simulink model "tp_thyr_rect_sm"  (R2026a)
settings: Solver=daessc  StopTime=simlength  FixedStep=Ts  MaxStep=Ts  RelTol=Ts  AbsTol=Ts  EnableMultiTasking=on
values from neighbouring files (symbols this model uses):
  I_FS = Iout_dc_nom * margin_factor    (= 103.5)    [init_model.m]
  kgrid = 1    [init_model.m]
  LFu_dc = 1.2e-3    (= 0.0012)    [init_model.m]
  pll_i1 = 80    [init_model.m]
  pll_p = 1    [init_model.m]
  RLFu_dc = 2e-4    (= 0.0002)    [init_model.m]
  Rload = 1.2/4    (= 0.3)    [init_model.m]
  Tc = 1e-5    (= 1e-05)    [init_model.m]
  Tcontrol_rect = tPWM_RECT    (= 0.0002)    [init_model.m]
  Ts = Tc/1    (= 1e-05)    [init_model.m]
  V_FS = Vout_dc_nom * margin_factor    (= 391)    [init_model.m]
  Vnom_ac_adc = 400/sqrt(3)*sqrt(2)    [init_model.m]
  Vphase1 = Vline1/sqrt(3)    [init_model.m]
  w_grid = f_grid*2*pi    (= 314.159265359)    [init_model.m]
undefined symbols (not defined in the file or in its folder): magnitude
libraries: fl_lib x248, nesl_utility x39, ee_lib x28
(part 1 of 5)
settings Model: Creator=LTNBDA  LastModifiedBy=dbagn
settings SolverCC: ZeroCrossControl=EnableAll  ZeroCrossAlgorithm=Adaptive  SolverResetMethod=Robust
settings DataIOCC: MaxDataPoints=1  SignalLoggingSaveFormat=ModelDataLogs
settings OptimizationCC: InitFltsAndDblsToZero=on  EfficientMapNaN2IntZero=off
settings DebuggingCC: SaveWithParameterizedLinksMsg=none  UnderspecifiedInitializationDetection=Classic  SignalResolutionControl=TryResolveAllWithWarning  MultiTaskDSMMsg=warning  MultiTaskCondExecSysMsg=none
settings HardwareCC: ProdBitPerLong=64.0  ProdHWDeviceType=Generic->64-bit Embedded Processor (LP64)  TargetBitPerPointer=64.0  TargetBitPerSizeT=64.0  TargetBitPerPtrDiffT=64.0  TargetLongLongMode=on  TargetIntDivRoundTo=Zero  TargetEndianess=LittleEndian  TargetWordSize=64.0  TargetHWDeviceType=MATLAB Host  ProdEqTarget=off
settings SFSimCC: SimCustomHeaderCode="#include \"twelve_pulse_rect.h\""  SimUserSources=src/twelve_pulse_rect.c  SimUserIncludeDirs=include
settings CodeAppCC: MaxIdLength=128.0
settings GRTTargetCC: CombineOutputUpdateFcns=off  GRTInterface=on
settings SimscapeCC: SimscapeNormalizeSystem=off  SimscapeNominalValues="[{\"value\":\"1\",\"unit\":\"A\"},{\"value\":\"1\",\"unit\":\"bar\"},{\"value\":\"1\",\"unit\":\"cm^2\"},{\"value\":\"1\",\"unit\":\"cm^3/s\"},{\"value\":\"1\",\"unit\":\"kJ/kg\"},{\"value\":\"1\",\"unit\":\"kW\"},{\"value\":\"1\",\"unit\":\"l\"},{\"value\":\"1\",\"unit\":\"N\"},{\"value\":\"1\",\"unit\":\"N*m\"},{\"value\":\"1\",\"unit\":\"V\"}]"  SimscapeLogType=none  SimscapeLogDataHistory=5000.0

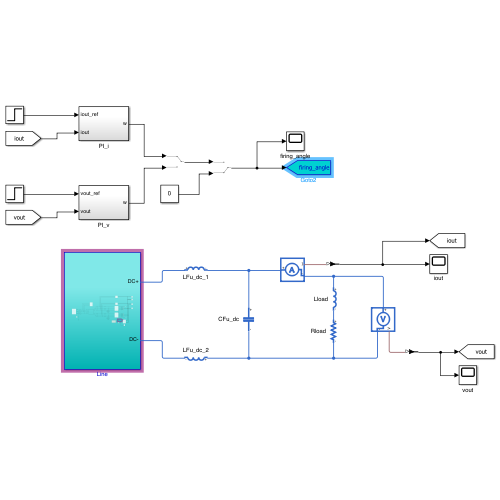
[thumbnail: Simulink's stored preview of the top-level diagram]
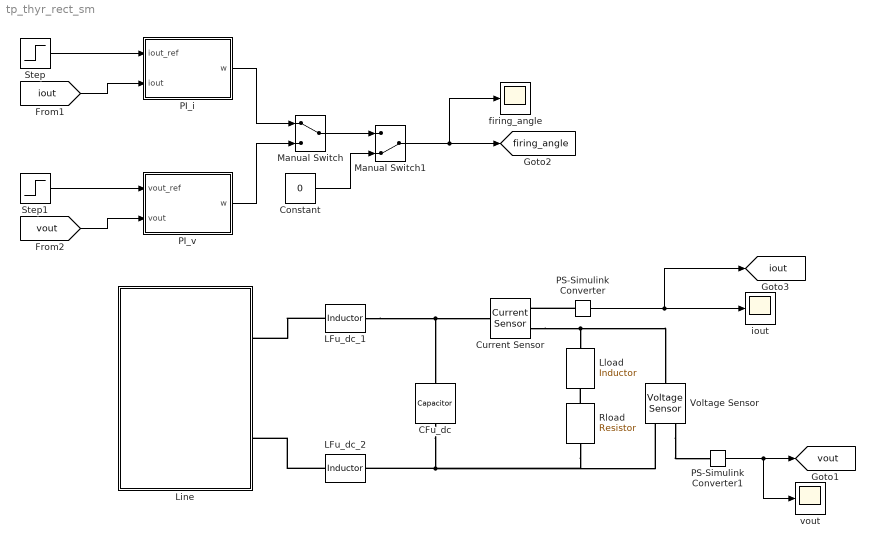
== system tp_thyr_rect_sm ==
  CFu_dc : fl_lib/Electrical/Electrical Elements/Capacitor  c=CFu_dc F  r=RCFu_dc Ohm  g=0 1/Ohm  i_specify=off  i_priority=None  i=0 A  i_nominal_specify=off  i_nominal_value=1  i_nominal_unit=A  v_specify=off  v_priority=None  v=0 V  v_nominal_specify=off  v_nominal_value=1  v_nominal_unit=V  vc_specify=off  vc_priority=High  vc=0 V  vc_nominal_specify=off  vc_nominal_value=1  vc_nominal_unit=V
  Constant : Constant  Value=0
  Current Sensor : fl_lib/Electrical/Electrical Sensors/Current Sensor
  LFu_dc_1 : fl_lib/Electrical/Electrical Elements/Inductor  l=LFu_dc/2 H  r=RLFu_dc/2 Ohm  g=1e-9 1/Ohm  i_specify=off  i_priority=None  i=0 A  i_nominal_specify=off  i_nominal_value=1  i_nominal_unit=A  v_specify=off  v_priority=None  v=0 V  v_nominal_specify=off  v_nominal_value=1  v_nominal_unit=V  i_L_specify=off  i_L_priority=High  i_L=0 A  i_L_nominal_specify=off  i_L_nominal_value=1  i_L_nominal_unit=A
  LFu_dc_2 : fl_lib/Electrical/Electrical Elements/Inductor  l=LFu_dc/2 H  r=RLFu_dc/2 Ohm  g=1e-9 1/Ohm  i_specify=off  i_priority=None  i=0 A  i_nominal_specify=off  i_nominal_value=1  i_nominal_unit=A  v_specify=off  v_priority=None  v=0 V  v_nominal_specify=off  v_nominal_value=1  v_nominal_unit=V  i_L_specify=off  i_L_priority=High  i_L=0 A  i_L_nominal_specify=off  i_L_nominal_value=1  i_L_nominal_unit=A
  Line : Subsystem
  Lload : fl_lib/Electrical/Electrical Elements/Inductor  l=Lload H  r=0 Ohm  g=1e-9 1/Ohm  i_specify=off  i_priority=None  i=0 A  i_nominal_specify=off  i_nominal_value=1  i_nominal_unit=A  v_specify=off  v_priority=None  v=0 V  v_nominal_specify=off  v_nominal_value=1  v_nominal_unit=V  i_L_specify=off  i_L_priority=High  i_L=0 A  i_L_nominal_specify=off  i_L_nominal_value=1  i_L_nominal_unit=A
  Manual Switch : ManualSwitch
  Manual Switch1 : ManualSwitch  CurrentSetting=0
  PI_i : Subsystem
  PI_v : Subsystem
  PS-Simulink Converter : nesl_utility/PS-Simulink Converter  PhysicalDomain=network_engine_domain  SubClassName=ps_output  LeftPortType=input  RightPortType=output  PseudoPeriodic=off  Frequencies=[]  VectorFormat=1-D array  Unit=A  AffineConversion=off
  PS-Simulink Converter1 : nesl_utility/PS-Simulink Converter  PhysicalDomain=network_engine_domain  SubClassName=ps_output  LeftPortType=input  RightPortType=output  PseudoPeriodic=off  Frequencies=[]  VectorFormat=1-D array  Unit=V  AffineConversion=on
  Rload : fl_lib/Electrical/Electrical Elements/Resistor  R=Rload Ohm  i_specify=off  i_priority=None  i=0 A  i_nominal_specify=off  i_nominal_value=1  i_nominal_unit=A  v_specify=off  v_priority=None  v=0 V  v_nominal_specify=off  v_nominal_value=1  v_nominal_unit=V
  Step : Step  Time=0.5  FinalValue=400/I_FS  SampleTime=0
  Step1 : Step  Time=0.5  FinalValue=400/V_FS  SampleTime=0
  Voltage Sensor : fl_lib/Electrical/Electrical Sensors/Voltage Sensor
  firing_angle : Scope
      settings: ActiveDisplayYMinimum=-11.249999999999998  ActiveDisplayYMaximum=101.25  DataLoggingVariableName=ScopeData5
  iout : Scope
      settings: SampleTime=Tcontrol_rect  ActiveDisplayYMinimum=-131.08083852559926  ActiveDisplayYMaximum=1179.7275467303937  DataLoggingVariableName=ScopeData10
  vout : Scope
      settings: SampleTime=Tcontrol_rect  ActiveDisplayYMinimum=-99.120870980483161  ActiveDisplayYMaximum=25.432476802314902
  tag scope: firing_angle=global, iout=global, vout=global
  wires:
  PS-Simulink Converter/1 -> [iout], iout/1
  Step/1 -> PI_i/1(iout_ref)
  PS-Simulink Converter1/1 -> vout/1, [vout]
  [iout] -> PI_i/2(iout)
  [vout] -> PI_v/2(vout)
  Step1/1 -> PI_v/1(vout_ref)
  PI_i/1(w) -> Manual Switch/1
  PI_v/1(w) -> Manual Switch/2
  Manual Switch/1 -> Manual Switch1/1
  Manual Switch1/1 -> firing_angle/1, [firing_angle]
  Constant/1 -> Manual Switch1/2
  connections:
  LFu_dc_1/RConn1 -- CFu_dc/LConn1 -- Current Sensor/LConn1
  CFu_dc/RConn1 -- Rload/RConn1 -- Voltage Sensor/RConn2 -- LFu_dc_2/LConn1
  LFu_dc_2/RConn1 -- Line/RConn2
  LFu_dc_1/LConn1 -- Line/RConn1
  Rload/LConn1 -- Lload/RConn1
  PS-Simulink Converter/LConn1 -- Current Sensor/RConn1
  Current Sensor/RConn2 -- Lload/LConn1 -- Voltage Sensor/LConn1
  Voltage Sensor/RConn1 -- PS-Simulink Converter1/LConn1

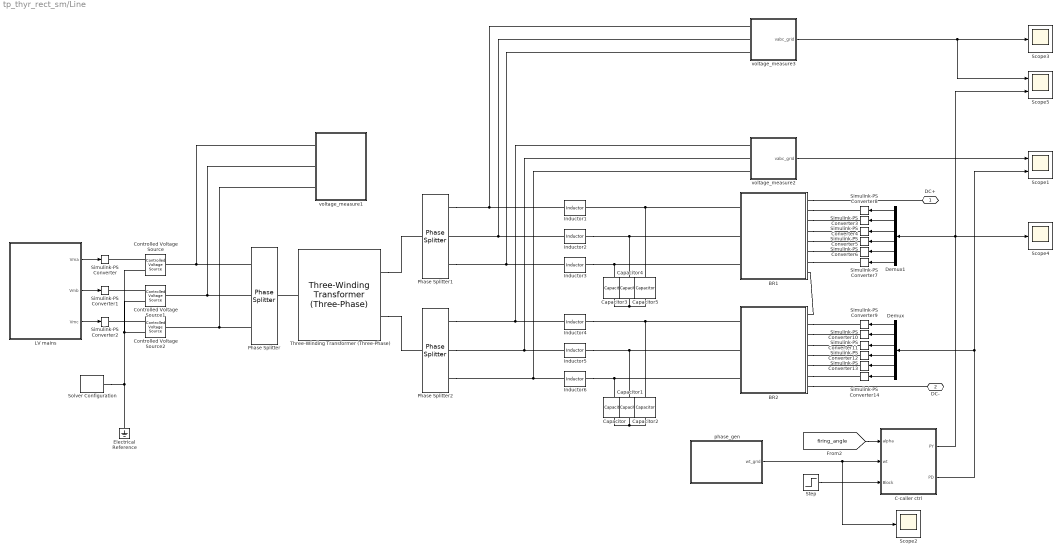
== system tp_thyr_rect_sm/Line ==
  BR1 : Subsystem
  BR2 : Subsystem
  C-caller ctrl : Subsystem
  Capacitor{,1..5} (6 alike) : fl_lib/Electrical/Electrical Elements/Capacitor  c=400e-6 F  r=1e-6 Ohm  g=0 1/Ohm  i_specify=off  i_priority=None  i=0 A  i_nominal_specify=off  i_nominal_value=1  i_nominal_unit=A  v_specify=off  v_priority=None  v=0 V  v_nominal_specify=off  v_nominal_value=1  v_nominal_unit=V  vc_specify=off  vc_priority=High  vc=0 V  vc_nominal_specify=off  vc_nominal_value=1  vc_nominal_unit=V
  Controlled Voltage Source : fl_lib/Electrical/Electrical Sources/Controlled Voltage Source
  Controlled Voltage Source1 : fl_lib/Electrical/Electrical Sources/Controlled Voltage Source
  Controlled Voltage Source2 : fl_lib/Electrical/Electrical Sources/Controlled Voltage Source
  Demux : Demux  Outputs=6
  Demux1 : Demux  Outputs=6
  Electrical Reference : fl_lib/Electrical/Electrical Elements/Electrical Reference
  Inductor{1..6} (6 alike) : fl_lib/Electrical/Electrical Elements/Inductor  l=500e-6 H  r=0 Ohm  g=1e-9 1/Ohm  i_specify=off  i_priority=None  i=0 A  i_nominal_specify=off  i_nominal_value=1  i_nominal_unit=A  v_specify=off  v_priority=None  v=0 V  v_nominal_specify=off  v_nominal_value=1  v_nominal_unit=V  i_L_specify=off  i_L_priority=High  i_L=0 A  i_L_nominal_specify=off  i_L_nominal_value=1  i_L_nominal_unit=A
  LV mains : Subsystem
  Phase Splitter : ee_lib/Connectors & References/Phase Splitter
  Phase Splitter1 : ee_lib/Connectors & References/Phase Splitter
  Phase Splitter2 : ee_lib/Connectors & References/Phase Splitter
  Scope1 : Scope  NumInputPorts=2
      settings: SampleTime=Tcontrol_rect  ActiveDisplayYMinimum=-1.2499074589151811  ActiveDisplayYMaximum=1.2499644999858517
  Scope2 : Scope
      settings: SampleTime=Tcontrol_rect  ActiveDisplayYMinimum=-0.60157607791225409  ActiveDisplayYMaximum=6.7110739220877456
  Scope3 : Scope
      settings: SampleTime=Tcontrol_rect  ActiveDisplayYMinimum=-0.5972  ActiveDisplayYMaximum=0.56165
  Scope4 : Scope
      settings: SampleTime=Tcontrol_rect  ActiveDisplayYMinimum=-1.4999999999999996  ActiveDisplayYMaximum=13.5
  Scope5 : Scope  NumInputPorts=2
      settings: SampleTime=Tcontrol_rect  ActiveDisplayYMinimum=-1.1962848065431293  ActiveDisplayYMaximum=1.2412506621236479  DataLoggingVariableName=ScopeData6
  Simulink-PS Converter{,1..3,5..10,12..14} (13 alike) : nesl_utility/Simulink-PS Converter  PhysicalDomain=network_engine_domain  SubClassName=ps_input  LeftPortType=input  RightPortType=output  PseudoPeriodic=off  Frequencies=[]  NoiseDistribution=none  NoiseParameters=[]  Unit=V  AffineConversion=on  FilteringAndDerivatives=provide  SimscapeFilterOrder=1  InputFilterTimeConstant=0.001  UdotUserProvided=0
  Simulink-PS Converter11 : nesl_utility/Simulink-PS Converter  PhysicalDomain=network_engine_domain  SubClassName=ps_input  LeftPortType=input  RightPortType=output  PseudoPeriodic=off  Frequencies=[]  NoiseDistribution=none  NoiseParameters=[]  Unit=V  AffineConversion=off  FilteringAndDerivatives=provide  SimscapeFilterOrder=1  InputFilterTimeConstant=0.001  UdotUserProvided=0
  Simulink-PS Converter4 : nesl_utility/Simulink-PS Converter  PhysicalDomain=network_engine_domain  SubClassName=ps_input  LeftPortType=input  RightPortType=output  PseudoPeriodic=off  Frequencies=[]  NoiseDistribution=none  NoiseParameters=[]  Unit=V  AffineConversion=off  FilteringAndDerivatives=provide  SimscapeFilterOrder=1  InputFilterTimeConstant=0.001  UdotUserProvided=0
  Solver Configuration : nesl_utility/Solver Configuration  PhysicalDomain=network_engine_domain  SubClassName=solver  LeftPortType=input  RightPortType=generic  Tones=[]  Harmonics=[]  SimulateNoise=off  Profile=off  UseLocalSampling=off  EnableSwitchedLinearOptims=on  FrequencyDomain=off  UseCCode=off  RelTol=0.001  AbsTol=1e-06  MinStep=1e-09  ToWorkspace=off  RevertToSquareIcSolve=off  NumHomotopyIterations=100  PhasorMode=off  PhasorModeNumHarmonics=1  ConsistencySolver=NEWTON_FTOL  CanonicalOrdering=UNORDERED  OptimizeIntermediates=UNOPTIMIZED  IndexReductionMethod=DerivativeReplacement  DoDC=off  ResidualTolerance=1e-09  ConsistencyTolSource=GLOBAL  ConsistencyAbsTol=0.001  ConsistencyRelTol=0.001  ConsistencyTolFactor=0.001  UseLocalSolver=on  LocalSolverChoice=NE_BACKWARD_EULER_ADVANCER  ResolveIndetEquations=on  FunctionEvalNumThread=1  LocalSolverSampleTime=Tcontrol_rect  DoFixedCost=on  MaxNonlinIter=3  MaxModeIter=2  ComputeImpulses=off  ImpulseIterations=2  LinearAlgebra=auto  LinearAlgebraNumThread=0  EquationFormulation=NE_TIME_EF  DelaysMemoryBudget=1024  AutomaticFiltering=on  FilteringTimeConstant=0.001  PartitionStorageMethod=AS_NEEDED  PartitionMemoryBudget=1024  PartitionMethod=ROBUST  MultibodyUseLocalSolver=off  MultibodyLocalSolverChoice=ODE1  MultibodyLocalSolverSampleTime=0.001
  Step : Step  Time=0.25  InitialValue=1  FinalValue=0  SampleTime=Tcontrol_rect
  Three-Winding Transformer (Three-Phase) : ee_lib/Passive/Transformers/Three-Winding Transformer (Three-Phase)  SRated=Pb V*A  FRated=50 Hz  Winding1Connection=ee.enum.windingconnection.Y  VRated1=V1b V  Winding2Connection=ee.enum.windingconnection.Y  VRated2=V2b V  Winding3Connection=ee.enum.windingconnection.delta1  VRated3=V2b V  CoreType=ee.enum.coretype.threelimb  pu_Rw1=r1pu  pu_Rw2=r2pu  pu_Rw3=r2pu  leakage_reactance_option=ee.enum.transformer_leakage.include  pu_Xl1=l1pu  pu_Xl2=l2pu  pu_Xl3=l2pu  magnetizing_resistance_option=ee.enum.transformer_magnetizingResistance.include  pu_Rm=500  magnetizing_reactance_option=ee.enum.transformer_magnetizingReactance.include  saturation_option=ee.enum.transformer_saturation.exclude  pu_Xm=500  current_data=[0, .002, 1, 2]  magnetic_flux_data=[0, 1.2, 1.5, 1.51]  pu_X0=0.5  i1_specify=off  i1_priority=None  i1=[ 0 0 0 ] A  i1_nominal_specify=off  i1_nominal_value=1  i1_nominal_unit=A  i2_specify=off  i2_priority=None  i2=[ 0 0 0 ] A  i2_nominal_specify=off  i2_nominal_value=1  i2_nominal_unit=A  i3_specify=off  i3_priority=None  i3=[ 0 0 0 ] A  i3_nominal_specify=off  i3_nominal_value=1  i3_nominal_unit=A  phi_specify=off  phi_priority=None  phi=[ 0 0 0 ]  phi_nominal_specify=off  phi_nominal_value=1  phi_nominal_unit=1
  phase_gen : Subsystem
  voltage_measure1 : Subsystem
  voltage_measure2 : Subsystem
  voltage_measure3 : Subsystem
  DC+ : PMIOPort  Side=Right
  DC- : PMIOPort  Port=2  Side=Right
  wires:
  [firing_angle] -> C-caller ctrl/1(alpha)
  phase_gen/1(wt_grid) -> Scope2/1, C-caller ctrl/2(wt)
  voltage_measure2/1(vabc_grid) -> Scope1/1
  Step/1 -> C-caller ctrl/3(Block)
  voltage_measure3/1(vabc_grid) -> Scope3/1, Scope5/1
  LV mains/1(Vma) -> Simulink-PS Converter/1
  LV mains/2(Vmb) -> Simulink-PS Converter1/1
  LV mains/3(Vmc) -> Simulink-PS Converter2/1
  Demux/1 -> Simulink-PS Converter9/1
  Demux/2 -> Simulink-PS Converter10/1
  Demux/3 -> Simulink-PS Converter11/1
  Demux/4 -> Simulink-PS Converter12/1
  Demux/5 -> Simulink-PS Converter13/1
  Demux/6 -> Simulink-PS Converter14/1
  Demux1/6 -> Simulink-PS Converter7/1
  Demux1/5 -> Simulink-PS Converter6/1
  Demux1/4 -> Simulink-PS Converter5/1
  Demux1/3 -> Simulink-PS Converter4/1
  Demux1/2 -> Simulink-PS Converter3/1
  Demux1/1 -> Simulink-PS Converter8/1
  C-caller ctrl/1(PY) -> Scope5/2, Demux1/1, Scope4/1
  C-caller ctrl/2(PD) -> Scope1/2, Demux/1
  connections:
  Controlled Voltage Source/RConn1 -- Simulink-PS Converter/RConn1
  Controlled Voltage Source1/RConn1 -- Simulink-PS Converter1/RConn1
  Controlled Voltage Source2/RConn1 -- Simulink-PS Converter2/RConn1
  Phase Splitter/RConn1 -- voltage_measure1/LConn1 -- Controlled Voltage Source/LConn1
  Phase Splitter/RConn2 -- voltage_measure1/LConn2 -- Controlled Voltage Source1/LConn1
  Phase Splitter/RConn3 -- voltage_measure1/LConn3 -- Controlled Voltage Source2/LConn1
  Three-Winding Transformer (Three-Phase)/LConn1 -- Phase Splitter/LConn1
  Three-Winding Transformer (Three-Phase)/RConn1 -- Phase Splitter1/LConn1
  Three-Winding Transformer (Three-Phase)/RConn2 -- Phase Splitter2/LConn1
  voltage_measure3/LConn2 -- Inductor2/LConn1 -- Phase Splitter1/RConn2
  Phase Splitter1/RConn3 -- Inductor3/LConn1 -- voltage_measure3/LConn3
  BR1/RConn1 -- Capacitor5/LConn1 -- Inductor1/RConn1
  BR2/RConn1 -- Inductor4/RConn1 -- Capacitor2/LConn1
  Phase Splitter2/RConn2 -- Inductor5/LConn1 -- voltage_measure2/LConn2
  Phase Splitter2/RConn3 -- Inductor6/LConn1 -- voltage_measure2/LConn3
  BR1/LConn1 -- DC+/RConn1
  BR2/LConn8 -- DC-/RConn1
  Controlled Voltage Source2/RConn2 -- Controlled Voltage Source1/RConn2 -- Controlled Voltage Source/RConn2 -- Solver Configuration/RConn1 -- Electrical Reference/LConn1
  BR2/LConn2 -- Simulink-PS Converter9/RConn1
  BR2/LConn3 -- Simulink-PS Converter10/RConn1
  BR2/LConn4 -- Simulink-PS Converter11/RConn1
  BR2/LConn5 -- Simulink-PS Converter12/RConn1
  BR2/LConn6 -- Simulink-PS Converter13/RConn1
  BR2/LConn7 -- Simulink-PS Converter14/RConn1
  BR1/LConn2 -- Simulink-PS Converter8/RConn1
  BR1/LConn3 -- Simulink-PS Converter3/RConn1
  BR1/LConn4 -- Simulink-PS Converter4/RConn1
  BR1/LConn5 -- Simulink-PS Converter5/RConn1
  BR1/LConn6 -- Simulink-PS Converter6/RConn1
  BR1/LConn7 -- Simulink-PS Converter7/RConn1
  BR2/LConn1 -- BR1/LConn8
  Inductor1/LConn1 -- Phase Splitter1/RConn1 -- voltage_measure3/LConn1
  BR1/RConn2 -- Inductor2/RConn1 -- Capacitor4/LConn1
  BR1/RConn3 -- Inductor3/RConn1 -- Capacitor3/LConn1
  voltage_measure2/LConn1 -- Inductor4/LConn1 -- Phase Splitter2/RConn1
  BR2/RConn2 -- Inductor5/RConn1 -- Capacitor1/LConn1
  BR2/RConn3 -- Inductor6/RConn1 -- Capacitor/LConn1
  Capacitor/RConn1 -- Capacitor1/RConn1 -- Capacitor2/RConn1
  Capacitor3/RConn1 -- Capacitor4/RConn1 -- Capacitor5/RConn1

== system tp_thyr_rect_sm/PI_i ==
  iout_ref : Inport
  iout : Inport  Port=2
  1/Ti : Gain  Gain=0.15  SaturateOnIntegerOverflow=on  OutDataTypeStr=Inherit: Same as input  ParamDataTypeStr=Inherit: Same as input
  1/Ti1 : Gain  Gain=180/pi  SaturateOnIntegerOverflow=on  OutDataTypeStr=Inherit: Same as input  ParamDataTypeStr=Inherit: Same as input
  1/Ti2 : Gain  Gain=1/I_FS  SaturateOnIntegerOverflow=on  OutDataTypeStr=Inherit: Same as input  ParamDataTypeStr=Inherit: Same as input
  Saturation : Saturate  UpperLimit=180  LowerLimit=0
  Saturation1 : Saturate  UpperLimit=1  LowerLimit=-1
  Sum1 : Sum  Inputs=+++  SaturateOnIntegerOverflow=on
  Sum2 : Sum  Inputs=+-  SaturateOnIntegerOverflow=on
  Sum3 : Sum  Inputs=-+  SaturateOnIntegerOverflow=on
  Trigonometric Function : Trigonometry  Operator=acos
  Unit Delay1 : UnitDelay  SampleTime=Tcontrol_rect
  Unit Delay4 : UnitDelay  SampleTime=Tcontrol_rect
  kp : Gain  Gain=8*Tcontrol_rect  SaturateOnIntegerOverflow=on  OutDataTypeStr=Inherit: Same as input  ParamDataTypeStr=Inherit: Same as input
  w : Outport  VectorParamsAs1DForOutWhenUnconnected=off
  wires:
  Sum2/1 -> 1/Ti/1, kp/1
  kp/1 -> Sum1/2
  1/Ti/1 -> Sum3/1, Sum1/1
  Unit Delay4/1 -> Sum1/3
  Sum3/1 -> Unit Delay4/1
  Sum1/1 -> Saturation1/1
  Trigonometric Function/1 -> 1/Ti1/1
  Saturation/1 -> Unit Delay1/1
  iout/1 -> 1/Ti2/1
  iout_ref/1 -> Sum2/1
  1/Ti2/1 -> Sum2/2
  Unit Delay1/1 -> w/1
  Saturation1/1 -> Sum3/2, Trigonometric Function/1
  1/Ti1/1 -> Saturation/1

== system tp_thyr_rect_sm/PI_v ==
  vout_ref : Inport
  vout : Inport  Port=2
  1/Ti : Gain  Gain=0.15  SaturateOnIntegerOverflow=on  OutDataTypeStr=Inherit: Same as input  ParamDataTypeStr=Inherit: Same as input
  1/Ti1 : Gain  Gain=180/pi  SaturateOnIntegerOverflow=on  OutDataTypeStr=Inherit: Same as input  ParamDataTypeStr=Inherit: Same as input
  1/Ti2 : Gain  Gain=1/V_FS  SaturateOnIntegerOverflow=on  OutDataTypeStr=Inherit: Same as input  ParamDataTypeStr=Inherit: Same as input
  Saturation : Saturate  UpperLimit=180  LowerLimit=0
  Saturation1 : Saturate  UpperLimit=1  LowerLimit=-1
  Sum1 : Sum  Inputs=+++  SaturateOnIntegerOverflow=on
  Sum2 : Sum  Inputs=+-  SaturateOnIntegerOverflow=on
  Sum3 : Sum  Inputs=-+  SaturateOnIntegerOverflow=on
  Trigonometric Function : Trigonometry  Operator=acos
  Unit Delay1 : UnitDelay  SampleTime=Tcontrol_rect
  Unit Delay4 : UnitDelay  SampleTime=Tcontrol_rect
  kp : Gain  Gain=8*Tcontrol_rect  SaturateOnIntegerOverflow=on  OutDataTypeStr=Inherit: Same as input  ParamDataTypeStr=Inherit: Same as input
  w : Outport  VectorParamsAs1DForOutWhenUnconnected=off
  wires:
  1/Ti1/1 -> Saturation/1
  Saturation1/1 -> Trigonometric Function/1, Sum3/2
  Unit Delay1/1 -> w/1
  1/Ti2/1 -> Sum2/2
  vout_ref/1 -> Sum2/1
  vout/1 -> 1/Ti2/1
  Saturation/1 -> Unit Delay1/1
  Trigonometric Function/1 -> 1/Ti1/1
  Sum1/1 -> Saturation1/1
  Sum3/1 -> Unit Delay4/1
  Unit Delay4/1 -> Sum1/3
  1/Ti/1 -> Sum1/1, Sum3/1
  kp/1 -> Sum1/2
  Sum2/1 -> kp/1, 1/Ti/1

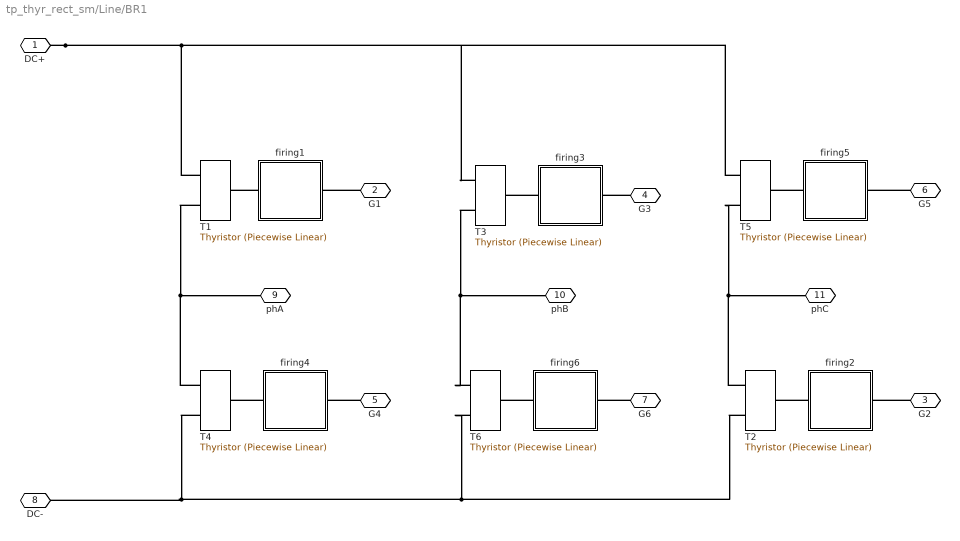
== system tp_thyr_rect_sm/Line/BR1 ==
  T{1..6} (6 alike) : ee_lib/Semiconductors & Converters/Thyristor (Piecewise Linear)  port_option=ee.enum.controlport.ps  Vf=0.8 V  Ron=0.001 Ohm  Goff=1e-5 1/Ohm  Vgt=6 V  Ih=1 A  diode_param=ee.enum.semiconductors.protectionDiode.nodynamics  diode_Vf=0.8 V  diode_Ron=0.001 Ohm  diode_Goff=1e-5 1/Ohm  diode_C=50e-9 F  diode_iRM=-235 A  diode_iF=300 A  diode_idot=-50 A/us  diode_trr_param=1  diode_trr_factor=3  diode_trr=15 us  diode_Qrr=1500 s*uA  iak_specify=off  iak_priority=None  iak=0 A  iak_nominal_specify=off  iak_nominal_value=1  iak_nominal_unit=A  vak_specify=off  vak_priority=None  vak=0 V  vak_nominal_specify=off  vak_nominal_value=1  vak_nominal_unit=V  vgk_specify=off  vgk_priority=None  vgk=0 V  vgk_nominal_specify=off  vgk_nominal_value=1  vgk_nominal_unit=V  thermal_loss_option=2  Von_data=[0, 1.1, 1.3, 1.45, 1.75, 2.25, 2.7; 0, 1, 1.15, 1.35, 1.7, 2.35, 3] V  Tj=[298.15, 398.15] K  Iout_data=[0, 10, 50, 100, 200, 400, 600] A  Eon_data=[0, .29, 1.43, 2.86, 5.71, 13.14, 22.86; 0, .57, 2.63, 5.14, 10.29, 20.57, 30.29] * 1e-3 J  Tj_loss=[298.15, 398.15] K  Iout_data_loss=[0, .1, 1, 5, 10, 20, 40, 70, 100] A  Eon_scalar=22.86e-3 J  Eoff_natural_commutation=10e-3 J  Voff=300 V  Iout_scalar=600 A  onCurrentMeasDelay=1e-4 s  diodeModelType=ee.enum.converters.diodeModelType.pwl  diodeTableType=ee.enum.diode.tableType.IfMat  diode_IfMat=[.07, .12, .19, 1.75, 4.24, 7.32, 11.2; .16, .3, .72, 2.14, 4.02, 6.35, 9.12] A  diode_VfMat=[.9, 1.15, 1.25, 1.5, 1.75, 2.17, 2.6, 2.85; .58, .68, .75, 1.1, 1.38, 1.77, 2.27, 2.7] V  diode_TjVec=[25, 125] degC  diode_VfVec=[.5, .7, .9, 1.3, 1.7, 2.1, 2.5] V  diode_IfVec=[.1, .2, .5, 1, 2, 4, 7, 10] A  diode_rec_loss_model=ee.enum.diode.reverseRecoveryModel.fixed  diode_ErecVal=0 J  diode_scaleWithIandV=true  diode_ErecMat=zeros(2, 3) J  diode_TjrecVec=[298.15, 398.15] K  diode_IfrecVec=[.1, 1, 10] A  diode_IrecVal=10 A  diode_VrecVal=10 V  diode_tFilter=1 / 1000 / 100 s  thermal_network_parameterization=ee.enum.thermalNetworkTopology.external  Rth=[.08, .5] K/W  Rth_Cauer=[.08, .1, .5] K/W  Rth_Foster=[.08, .14, .22, .16] K/W  thermal_mass_parameterization=ee.enum.thermalNetwork.timeconstant  thermal_mass=[.01, .5] J/K  thermal_mass_Cauer=[.01, .1, .5] J/K  thermal_mass_Foster=[.001, .005, .05, .5] J/K  thermal_time_constant=[.001, .2] s  thermal_time_constant_Cauer=[.001, .1, .2] s  thermal_time_constant_Foster=[7e-05, .0007, .01, .08] s  thermal_mass_initial_temperatures=[25, 25] degC  thermal_mass_initial_temperatures_Cauer=[25, 25, 25] degC  junction_thermal_mass=0.01 J/K  Tvec_initial_Foster=[25, 25, 25, 25] degC  junction_temperature_specify=off  junction_temperature_priority=None  junction_temperature=25 degC  junction_temperature_nominal_specify=off  junction_temperature_nominal_value=1  junction_temperature_nominal_unit=degC  Qj_specify=off  Qj_priority=None  Qj=0 W  Qj_nominal_specify=off  Qj_nominal_value=1  Qj_nominal_unit=W  accumulatedSwitchingLosses_specify=off  accumulatedSwitchingLosses_priority=None  accumulatedSwitchingLosses=0 J
  firing1 : Subsystem
  firing2 : Subsystem
  firing3 : Subsystem
  firing4 : Subsystem
  firing5 : Subsystem
  firing6 : Subsystem
  DC+ : PMIOPort  Side=Left
  G1 : PMIOPort  Port=2  Side=Left
  G2 : PMIOPort  Port=3  Side=Left
  G3 : PMIOPort  Port=4  Side=Left
  G4 : PMIOPort  Port=5  Side=Left
  G5 : PMIOPort  Port=6  Side=Left
  G6 : PMIOPort  Port=7  Side=Left
  DC- : PMIOPort  Port=8  Side=Left
  phA : PMIOPort  Port=9  Side=Right
  phB : PMIOPort  Port=10  Side=Right
  phC : PMIOPort  Port=11  Side=Right
  connections:
  DC+/RConn1 -- T1/RConn2 -- T5/RConn2 -- T3/RConn2
  T4/RConn2 -- T1/RConn1 -- phA/RConn1
  T2/RConn2 -- T5/RConn1 -- phC/RConn1
  T3/RConn1 -- T6/RConn2 -- phB/RConn1
  T2/RConn1 -- T6/RConn1 -- T4/RConn1 -- DC-/RConn1
  G1/RConn1 -- firing1/LConn1
  G2/RConn1 -- firing2/LConn1
  G3/RConn1 -- firing3/LConn1
  G4/RConn1 -- firing4/LConn1
  G5/RConn1 -- firing5/LConn1
  G6/RConn1 -- firing6/LConn1
  firing2/RConn1 -- T2/LConn1
  firing3/RConn1 -- T3/LConn1
  firing4/RConn1 -- T4/LConn1
  firing5/RConn1 -- T5/LConn1
  firing6/RConn1 -- T6/LConn1
  firing1/RConn1 -- T1/LConn1

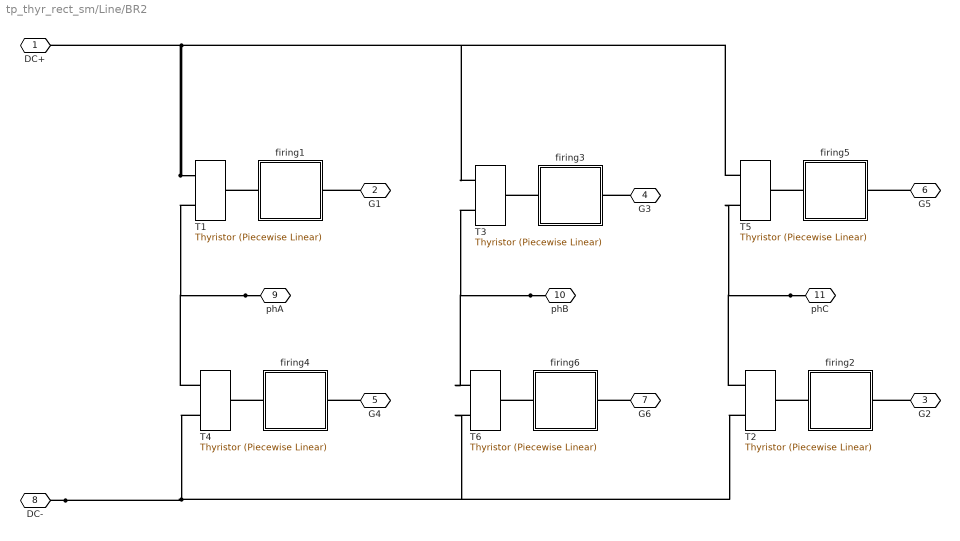
== system tp_thyr_rect_sm/Line/BR2 ==
  T{1..6} (6 alike) : ee_lib/Semiconductors & Converters/Thyristor (Piecewise Linear)  port_option=ee.enum.controlport.ps  Vf=0.8 V  Ron=0.001 Ohm  Goff=1e-5 1/Ohm  Vgt=6 V  Ih=1 A  diode_param=ee.enum.semiconductors.protectionDiode.nodynamics  diode_Vf=0.8 V  diode_Ron=0.001 Ohm  diode_Goff=1e-5 1/Ohm  diode_C=50e-9 F  diode_iRM=-235 A  diode_iF=300 A  diode_idot=-50 A/us  diode_trr_param=1  diode_trr_factor=3  diode_trr=15 us  diode_Qrr=1500 s*uA  iak_specify=off  iak_priority=None  iak=0 A  iak_nominal_specify=off  iak_nominal_value=1  iak_nominal_unit=A  vak_specify=off  vak_priority=None  vak=0 V  vak_nominal_specify=off  vak_nominal_value=1  vak_nominal_unit=V  vgk_specify=off  vgk_priority=None  vgk=0 V  vgk_nominal_specify=off  vgk_nominal_value=1  vgk_nominal_unit=V  thermal_loss_option=2  Von_data=[0, 1.1, 1.3, 1.45, 1.75, 2.25, 2.7; 0, 1, 1.15, 1.35, 1.7, 2.35, 3] V  Tj=[298.15, 398.15] K  Iout_data=[0, 10, 50, 100, 200, 400, 600] A  Eon_data=[0, .29, 1.43, 2.86, 5.71, 13.14, 22.86; 0, .57, 2.63, 5.14, 10.29, 20.57, 30.29] * 1e-3 J  Tj_loss=[298.15, 398.15] K  Iout_data_loss=[0, .1, 1, 5, 10, 20, 40, 70, 100] A  Eon_scalar=22.86e-3 J  Eoff_natural_commutation=10e-3 J  Voff=300 V  Iout_scalar=600 A  onCurrentMeasDelay=1e-4 s  diodeModelType=ee.enum.converters.diodeModelType.pwl  diodeTableType=ee.enum.diode.tableType.IfMat  diode_IfMat=[.07, .12, .19, 1.75, 4.24, 7.32, 11.2; .16, .3, .72, 2.14, 4.02, 6.35, 9.12] A  diode_VfMat=[.9, 1.15, 1.25, 1.5, 1.75, 2.17, 2.6, 2.85; .58, .68, .75, 1.1, 1.38, 1.77, 2.27, 2.7] V  diode_TjVec=[25, 125] degC  diode_VfVec=[.5, .7, .9, 1.3, 1.7, 2.1, 2.5] V  diode_IfVec=[.1, .2, .5, 1, 2, 4, 7, 10] A  diode_rec_loss_model=ee.enum.diode.reverseRecoveryModel.fixed  diode_ErecVal=0 J  diode_scaleWithIandV=true  diode_ErecMat=zeros(2, 3) J  diode_TjrecVec=[298.15, 398.15] K  diode_IfrecVec=[.1, 1, 10] A  diode_IrecVal=10 A  diode_VrecVal=10 V  diode_tFilter=1 / 1000 / 100 s  thermal_network_parameterization=ee.enum.thermalNetworkTopology.external  Rth=[.08, .5] K/W  Rth_Cauer=[.08, .1, .5] K/W  Rth_Foster=[.08, .14, .22, .16] K/W  thermal_mass_parameterization=ee.enum.thermalNetwork.timeconstant  thermal_mass=[.01, .5] J/K  thermal_mass_Cauer=[.01, .1, .5] J/K  thermal_mass_Foster=[.001, .005, .05, .5] J/K  thermal_time_constant=[.001, .2] s  thermal_time_constant_Cauer=[.001, .1, .2] s  thermal_time_constant_Foster=[7e-05, .0007, .01, .08] s  thermal_mass_initial_temperatures=[25, 25] degC  thermal_mass_initial_temperatures_Cauer=[25, 25, 25] degC  junction_thermal_mass=0.01 J/K  Tvec_initial_Foster=[25, 25, 25, 25] degC  junction_temperature_specify=off  junction_temperature_priority=None  junction_temperature=25 degC  junction_temperature_nominal_specify=off  junction_temperature_nominal_value=1  junction_temperature_nominal_unit=degC  Qj_specify=off  Qj_priority=None  Qj=0 W  Qj_nominal_specify=off  Qj_nominal_value=1  Qj_nominal_unit=W  accumulatedSwitchingLosses_specify=off  accumulatedSwitchingLosses_priority=None  accumulatedSwitchingLosses=0 J
  firing1 : Subsystem
  firing2 : Subsystem
  firing3 : Subsystem
  firing4 : Subsystem
  firing5 : Subsystem
  firing6 : Subsystem
  DC+ : PMIOPort  Side=Left
  G1 : PMIOPort  Port=2  Side=Left
  G2 : PMIOPort  Port=3  Side=Left
  G3 : PMIOPort  Port=4  Side=Left
  G4 : PMIOPort  Port=5  Side=Left
  G5 : PMIOPort  Port=6  Side=Left
  G6 : PMIOPort  Port=7  Side=Left
  DC- : PMIOPort  Port=8  Side=Left
  phA : PMIOPort  Port=9  Side=Right
  phB : PMIOPort  Port=10  Side=Right
  phC : PMIOPort  Port=11  Side=Right
  connections:
  firing6/RConn1 -- T6/LConn1
  firing5/RConn1 -- T5/LConn1
  firing4/RConn1 -- T4/LConn1
  firing3/RConn1 -- T3/LConn1
  firing2/RConn1 -- T2/LConn1
  firing1/RConn1 -- T1/LConn1
  G6/RConn1 -- firing6/LConn1
  G5/RConn1 -- firing5/LConn1
  G4/RConn1 -- firing4/LConn1
  G3/RConn1 -- firing3/LConn1
  G2/RConn1 -- firing2/LConn1
  G1/RConn1 -- firing1/LConn1
  DC-/RConn1 -- T4/RConn1 -- T6/RConn1 -- T2/RConn1
  phB/RConn1 -- T6/RConn2 -- T3/RConn1
  phC/RConn1 -- T5/RConn1 -- T2/RConn2
  phA/RConn1 -- T4/RConn2 -- T1/RConn1
  T1/RConn2 -- T3/RConn2 -- T5/RConn2 -- DC+/RConn1

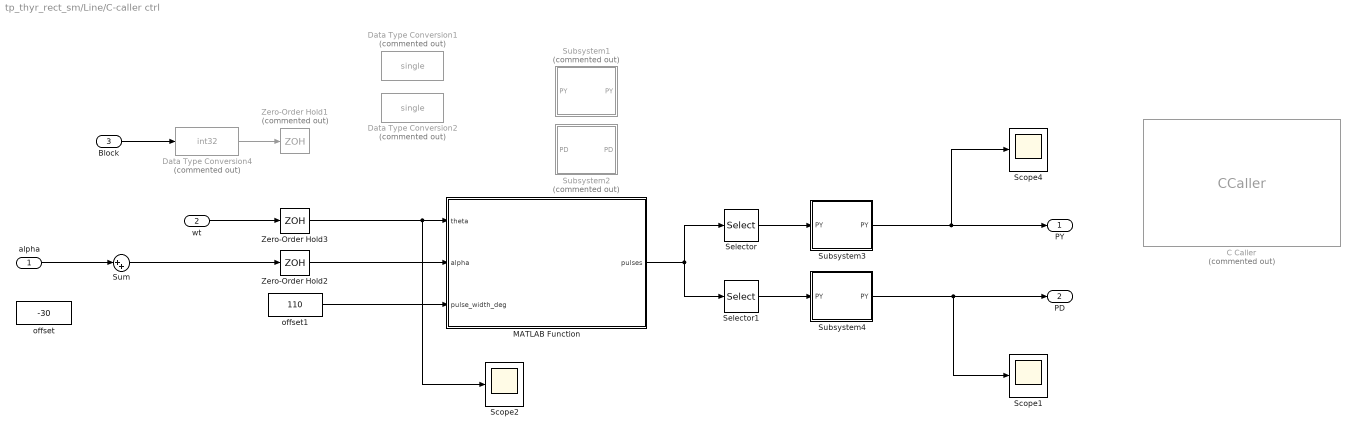
== system tp_thyr_rect_sm/Line/C-caller ctrl ==
  alpha : Inport  SampleTime=Ts
  wt : Inport  Port=2  SampleTime=Ts
  Block : Inport  Port=3  SampleTime=Ts
  C Caller : CCaller  Commented=on  FunctionName=twvprProcessSimulink  PortSpecificationStruct="%)30     .    R @   8    (     @         %    \"     4    !     0         %  0 \"0    $    _    07)G3F%M90  4&]R=$YA;64 4V-O<&4     26YD97@     5'EP90      4VEZ90      27-';&]B86P   X    P    !@    @    $          4    (     0    (    !         !   @!W=   #@   #     &    \"     0         !0    @    !     @    $         $  \" '=T   .    .     8    (    !          %    \"     $    %     0         0  ...(+2649 chars)"  SampleTime=Tcontrol_rect
  Data Type Conversion1 : DataTypeConversion  Commented=on  OutDataTypeStr=single  SaturateOnIntegerOverflow=off  RndMeth=Floor
  Data Type Conversion2 : DataTypeConversion  Commented=on  OutDataTypeStr=single  SaturateOnIntegerOverflow=off  RndMeth=Floor
  Data Type Conversion4 : DataTypeConversion  Commented=on  OutDataTypeStr=int32  SaturateOnIntegerOverflow=off  RndMeth=Floor
  MATLAB Function : MATLAB Function  TreatAsAtomicUnit=on
  Scope1 : Scope
      settings: SampleTime=Tcontrol_rect  ActiveDisplayYMinimum=-1.4999999999999996  ActiveDisplayYMaximum=13.5  DataLoggingVariableName=ScopeData3
  Scope2 : Scope
      settings: SampleTime=Tcontrol_rect  ActiveDisplayYMinimum=-0.77754418176338136  ActiveDisplayYMaximum=6.9978976358713938  DataLoggingVariableName=ScopeData4
  Scope4 : Scope
      settings: SampleTime=Tcontrol_rect  ActiveDisplayYMinimum=-1.4714285714285715  ActiveDisplayYMaximum=13.528571428571428  DataLoggingVariableName=ScopeData2
  Selector : Selector  InputPortWidth=12  IndexOptions=Index vector (dialog)  Indices=[1 2 3 4 5 6]  OutputSizes=1
  Selector1 : Selector  InputPortWidth=12  IndexOptions=Index vector (dialog)  Indices=[7 8 9 10 11 12]  OutputSizes=1
  Subsystem1 : Subsystem  Commented=on
  Subsystem2 : Subsystem  Commented=on
  Subsystem3 : Subsystem
  Subsystem4 : Subsystem
  Sum : Sum  Inputs=|++
  Zero-Order Hold1 : ZeroOrderHold  Commented=on  SampleTime=Tcontrol_rect
  Zero-Order Hold2 : ZeroOrderHold  SampleTime=Tcontrol_rect
  Zero-Order Hold3 : ZeroOrderHold  SampleTime=Tcontrol_rect
  offset : Constant  Value=-30  SampleTime=Ts
  offset1 : Constant  Value=110  SampleTime=Ts
  PY : Outport  SampleTime=Ts  InitialOutput=0  VectorParamsAs1DForOutWhenUnconnected=off
  PD : Outport  Port=2  SampleTime=Ts  InitialOutput=0  VectorParamsAs1DForOutWhenUnconnected=off
  wires:
  alpha/1 -> Sum/1
  Sum/1 -> Zero-Order Hold2/1
  wt/1 -> Zero-Order Hold3/1
  Data Type Conversion4/1 -> Zero-Order Hold1/1
  Zero-Order Hold3/1 -> MATLAB Function/1(theta), Scope2/1
  Zero-Order Hold2/1 -> MATLAB Function/2(alpha)
  offset1/1 -> MATLAB Function/3(pulse_width_deg)
  Block/1 -> Data Type Conversion4/1
  Selector/1 -> Subsystem3/1("PY ")
  Selector1/1 -> Subsystem4/1("PY ")
  MATLAB Function/1(pulses) -> Selector/1, Selector1/1
  Subsystem3/1(PY) -> Scope4/1, PY/1
  Subsystem4/1(PY) -> PD/1, Scope1/1

== system tp_thyr_rect_sm/Line/LV mains ==
  Clock : Clock
  Constant2 : Constant  Value=2*pi/3
  Constant3 : Constant  Value=4*pi/3
  Gain : Gain  Gain=w_grid
  Gain1 : Gain  Gain=Vphase1*sqrt(2)
  Gain2 : Gain  Gain=Vphase1*sqrt(2)
  Gain3 : Gain  Gain=Vphase1*sqrt(2)
  Gain4 : Gain  Gain=kgrid
  Gain5 : Gain  Gain=kgrid
  Gain6 : Gain  Gain=kgrid
  Sum2 : Sum  Inputs=+-|
  Sum3 : Sum  Inputs=+-|
  Trigonometric Function : Trigonometry  Operator=cos
  Trigonometric Function1 : Trigonometry  Operator=cos
  Trigonometric Function2 : Trigonometry  Operator=cos
  Vma : Outport
  Vmb : Outport  Port=2
  Vmc : Outport  Port=3
  wires:
  Trigonometric Function/1 -> Gain1/1
  Constant2/1 -> Sum2/2
  Sum2/1 -> Trigonometric Function1/1
  Constant3/1 -> Sum3/2
  Sum3/1 -> Trigonometric Function2/1
  Clock/1 -> Gain/1
  Gain/1 -> Sum3/1, Trigonometric Function/1, Sum2/1  "wt"
  Trigonometric Function1/1 -> Gain2/1
  Trigonometric Function2/1 -> Gain3/1
  Gain1/1 -> Gain4/1
  Gain2/1 -> Gain5/1
  Gain3/1 -> Gain6/1
  Gain4/1 -> Vma/1
  Gain5/1 -> Vmb/1
  Gain6/1 -> Vmc/1

== system tp_thyr_rect_sm/Line/phase_gen ==
  pll_stageA : Subsystem
  pll_stageB : Subsystem
  wt_grid : Outport
  wires:
  pll_stageA/1(Vgrid_a) -> pll_stageB/1(Vgrid_a)
  pll_stageA/2(Vgrid_b) -> pll_stageB/2(Vgrid_b)
  [vabc_grid_A] -> pll_stageA/1(VgridLL)
  pll_stageB/1(wt_grid) -> wt_grid/1

== system tp_thyr_rect_sm/Line/voltage_measure1 ==
  Gain1 : Gain  Gain=1/Vnom_ac_adc
  Gain2 : Gain  Gain=1/Vnom_ac_adc
  Gain3 : Gain  Gain=1/Vnom_ac_adc
  Gain4 : Gain  Gain=1/3
  Gain5 : Gain  Gain=1/3
  Gain6 : Gain  Gain=1/3
  Mux : Mux  Inputs=3
  PS-Simulink Converter : nesl_utility/PS-Simulink Converter  PhysicalDomain=network_engine_domain  SubClassName=ps_output  LeftPortType=input  RightPortType=output  PseudoPeriodic=off  Frequencies=[]  VectorFormat=1-D array  Unit=inherit  AffineConversion=off
  PS-Simulink Converter1 : nesl_utility/PS-Simulink Converter  PhysicalDomain=network_engine_domain  SubClassName=ps_output  LeftPortType=input  RightPortType=output  PseudoPeriodic=off  Frequencies=[]  VectorFormat=1-D array  Unit=inherit  AffineConversion=off
  PS-Simulink Converter2 : nesl_utility/PS-Simulink Converter  PhysicalDomain=network_engine_domain  SubClassName=ps_output  LeftPortType=input  RightPortType=output  PseudoPeriodic=off  Frequencies=[]  VectorFormat=1-D array  Unit=inherit  AffineConversion=off
  Sum : Sum  Inputs=|+-
  Sum1 : Sum  Inputs=|+-
  Sum2 : Sum  Inputs=|+-
  Voltage Sensor : fl_lib/Electrical/Electrical Sensors/Voltage Sensor
  Voltage Sensor1 : fl_lib/Electrical/Electrical Sensors/Voltage Sensor
  Voltage Sensor2 : fl_lib/Electrical/Electrical Sensors/Voltage Sensor
  va : PMIOPort  Side=Left
  vb : PMIOPort  Port=2  Side=Left
  vc : PMIOPort  Port=3  Side=Left
  tag scope: vabc_grid_A=global
  wires:
  Mux/1 -> [vabc_grid_A]
  PS-Simulink Converter/1 -> Gain1/1
  PS-Simulink Converter2/1 -> Gain3/1
  PS-Simulink Converter1/1 -> Gain2/1
  Gain6/1 -> Mux/3
  Gain4/1 -> Mux/1
  Gain5/1 -> Mux/2
  Gain1/1 -> Sum/1, Sum1/2
  Sum/1 -> Gain4/1
  Gain3/1 -> Sum2/1, Sum/2
  Sum1/1 -> Gain5/1
  Gain2/1 -> Sum2/2, Sum1/1
  Sum2/1 -> Gain6/1
  connections:
  Voltage Sensor/LConn1 -- Voltage Sensor2/RConn2 -- va/RConn1
  vb/RConn1 -- Voltage Sensor1/LConn1 -- Voltage Sensor/RConn2
  Voltage Sensor/RConn1 -- PS-Simulink Converter/LConn1
  Voltage Sensor1/RConn1 -- PS-Simulink Converter1/LConn1
  Voltage Sensor1/RConn2 -- Voltage Sensor2/LConn1 -- vc/RConn1
  Voltage Sensor2/RConn1 -- PS-Simulink Converter2/LConn1

== system tp_thyr_rect_sm/Line/voltage_measure2 ==
  note: // TENSIONI DI FASE LATO LINEA RICOSTUITE
      | 	param.u_grid_b = (param.u_grid_bc - param.u_grid_ab)/3;
      | 	param.u_grid_a = (param.u_grid_ab - param.u_grid_ca)/3;
      | 	param.u_grid_c = (param.u_grid_ca - param.u_grid_bc)/3;
  Gain1 : Gain  Gain=1/Vnom_ac_adc
  Gain2 : Gain  Gain=1/Vnom_ac_adc
  Gain3 : Gain  Gain=1/Vnom_ac_adc
  Gain4 : Gain  Gain=2/3
  Gain5 : Gain  Gain=2/3
  Gain6 : Gain  Gain=2/3
  Mux : Mux  Inputs=3
  PS-Simulink Converter : nesl_utility/PS-Simulink Converter  PhysicalDomain=network_engine_domain  SubClassName=ps_output  LeftPortType=input  RightPortType=output  PseudoPeriodic=off  Frequencies=[]  VectorFormat=1-D array  Unit=inherit  AffineConversion=off
  PS-Simulink Converter1 : nesl_utility/PS-Simulink Converter  PhysicalDomain=network_engine_domain  SubClassName=ps_output  LeftPortType=input  RightPortType=output  PseudoPeriodic=off  Frequencies=[]  VectorFormat=1-D array  Unit=inherit  AffineConversion=off
  PS-Simulink Converter2 : nesl_utility/PS-Simulink Converter  PhysicalDomain=network_engine_domain  SubClassName=ps_output  LeftPortType=input  RightPortType=output  PseudoPeriodic=off  Frequencies=[]  VectorFormat=1-D array  Unit=inherit  AffineConversion=off
  Sum : Sum  Inputs=|+-
  Sum1 : Sum  Inputs=|+-
  Sum2 : Sum  Inputs=|+-
  Voltage Sensor : fl_lib/Electrical/Electrical Sensors/Voltage Sensor
  Voltage Sensor1 : fl_lib/Electrical/Electrical Sensors/Voltage Sensor
  Voltage Sensor2 : fl_lib/Electrical/Electrical Sensors/Voltage Sensor
  va : PMIOPort  Side=Left
  vb : PMIOPort  Port=2  Side=Left
  vc : PMIOPort  Port=3  Side=Left
  vabc_grid : Outport
  wires:
  PS-Simulink Converter1/1 -> Gain2/1  "vbc"
  PS-Simulink Converter2/1 -> Gain3/1  "vca"
  PS-Simulink Converter/1 -> Gain1/1  "vab"
  Mux/1 -> vabc_grid/1
  Gain1/1 -> Sum1/2, Sum/1
  Gain3/1 -> Sum2/1, Sum/2
  Sum/1 -> Gain6/1
  Sum1/1 -> Gain4/1
  Sum2/1 -> Gain5/1
  Gain2/1 -> Sum2/2, Sum1/1
  Gain6/1 -> Mux/1
  Gain4/1 -> Mux/2
  Gain5/1 -> Mux/3
  connections:
  Voltage Sensor/RConn2 -- vb/RConn1 -- Voltage Sensor1/LConn1
  Voltage Sensor2/RConn2 -- va/RConn1 -- Voltage Sensor/LConn1
  Voltage Sensor/RConn1 -- PS-Simulink Converter/LConn1
  Voltage Sensor2/RConn1 -- PS-Simulink Converter2/LConn1
  Voltage Sensor1/RConn2 -- vc/RConn1 -- Voltage Sensor2/LConn1
  Voltage Sensor1/RConn1 -- PS-Simulink Converter1/LConn1

== system tp_thyr_rect_sm/Line/voltage_measure3 ==
  note: // TENSIONI DI FASE LATO LINEA RICOSTUITE
      | 	param.u_grid_b = (param.u_grid_bc - param.u_grid_ab)/3;
      | 	param.u_grid_a = (param.u_grid_ab - param.u_grid_ca)/3;
      | 	param.u_grid_c = (param.u_grid_ca - param.u_grid_bc)/3;
  Gain1 : Gain  Gain=1/Vnom_ac_adc
  Gain2 : Gain  Gain=1/Vnom_ac_adc
  Gain3 : Gain  Gain=1/Vnom_ac_adc
  Gain4 : Gain  Gain=2/3
  Gain5 : Gain  Gain=2/3
  Gain6 : Gain  Gain=2/3
  Mux : Mux  Inputs=3
  PS-Simulink Converter : nesl_utility/PS-Simulink Converter  PhysicalDomain=network_engine_domain  SubClassName=ps_output  LeftPortType=input  RightPortType=output  PseudoPeriodic=off  Frequencies=[]  VectorFormat=1-D array  Unit=inherit  AffineConversion=off
  PS-Simulink Converter1 : nesl_utility/PS-Simulink Converter  PhysicalDomain=network_engine_domain  SubClassName=ps_output  LeftPortType=input  RightPortType=output  PseudoPeriodic=off  Frequencies=[]  VectorFormat=1-D array  Unit=inherit  AffineConversion=off
  PS-Simulink Converter2 : nesl_utility/PS-Simulink Converter  PhysicalDomain=network_engine_domain  SubClassName=ps_output  LeftPortType=input  RightPortType=output  PseudoPeriodic=off  Frequencies=[]  VectorFormat=1-D array  Unit=inherit  AffineConversion=off
  Sum : Sum  Inputs=|+-
  Sum1 : Sum  Inputs=|+-
  Sum2 : Sum  Inputs=|+-
  Voltage Sensor : fl_lib/Electrical/Electrical Sensors/Voltage Sensor
  Voltage Sensor1 : fl_lib/Electrical/Electrical Sensors/Voltage Sensor
  Voltage Sensor2 : fl_lib/Electrical/Electrical Sensors/Voltage Sensor
  va : PMIOPort  Side=Left
  vb : PMIOPort  Port=2  Side=Left
  vc : PMIOPort  Port=3  Side=Left
  vabc_grid : Outport
  wires:
  Gain6/1 -> Mux/3
  Gain5/1 -> Mux/2
  Gain4/1 -> Mux/1
  Gain2/1 -> Sum1/1, Sum2/2
  Sum2/1 -> Gain6/1
  Sum1/1 -> Gain5/1
  Sum/1 -> Gain4/1
  Gain3/1 -> Sum/2, Sum2/1
  Gain1/1 -> Sum/1, Sum1/2
  Mux/1 -> vabc_grid/1
  PS-Simulink Converter/1 -> Gain1/1  "vab"
  PS-Simulink Converter2/1 -> Gain3/1  "vca"
  PS-Simulink Converter1/1 -> Gain2/1  "vbc"
  connections:
  Voltage Sensor1/RConn1 -- PS-Simulink Converter1/LConn1
  vc/RConn1 -- Voltage Sensor1/RConn2 -- Voltage Sensor2/LConn1
  Voltage Sensor2/RConn1 -- PS-Simulink Converter2/LConn1
  Voltage Sensor/RConn1 -- PS-Simulink Converter/LConn1
  va/RConn1 -- Voltage Sensor2/RConn2 -- Voltage Sensor/LConn1
  vb/RConn1 -- Voltage Sensor/RConn2 -- Voltage Sensor1/LConn1
